simulink model "pid_aw_lazo"  (R2025b)
settings: Solver=FixedStepDiscrete  StartTime=0.0  StopTime=10  FixedStep=Ts  RelTol=1e-3
PreLoadFcn:
  | Ts = 1e-3; tau = 0.01; ad = exp(-Ts/tau); bd = 1 - ad;
undefined symbols (not defined in the file or in its folder): dspblkCoreblockFVToolHelper, gcbh
settings Model: SILPILSystemUnderTest=refmodels  CodeVerificationMode=processor-in-the-loop (pil)  Creator=jnune  LastModifiedBy=jnune
settings OptimizationCC: DefaultParameterBehavior=Inlined  EnhancedBackFolding=on  PassReuseOutputArgsAs=Individual arguments  ZeroExternalMemoryAtStartup=off  ZeroInternalMemoryAtStartup=off  MaxStackSize=64  OptimizeBlockOrder=speed  DifferentSizesBufferReuse=on  OptimizationCustomize=off  EfficientTunableParamExpr=on
settings DebuggingCC: ParameterPrecisionLossMsg=none  ParameterTunabilityLossMsg=error
settings HardwareCC: ProdBitPerPointer=32.0  ProdBitPerSizeT=32.0  ProdBitPerPtrDiffT=32.0  ProdLargestAtomicInteger=Long  ProdLargestAtomicFloat=Double  ProdWordSize=32.0  ProdLongLongMode=on  ProdHWDeviceType=ARM Compatible->ARM Cortex-M
settings SFSimCC: MATLABDynamicMemAlloc=off
settings RTWCC: SystemTargetFile=ert.tlc  HardwareBoard=STM32 Nucleo F767ZI  TemplateMakefile=ert_default_tmf  Toolchain=GNU Tools for ARM Embedded Processors  CodeExecutionProfiling=on  CodeProfilingSaveOptions=AllData  Description=Embedded Coder
settings CodeAppCC: ForceParamTrailComments=on  IgnoreCustomStorageClasses=off  OperatorAnnotations=on  SimulinkDataObjDesc=on  SFDataObjDesc=on  InsertBlockDesc=on
settings ERTTargetCC: ExtModeTransport=3.0  ExtModeStaticAlloc=on  ExtModeStaticAllocSize=2000.0  ExtModeMexFile=ext_xcp  ExtModeIntrfLevel=Level2 - Open  TargetLangStandard=C99 (ISO)

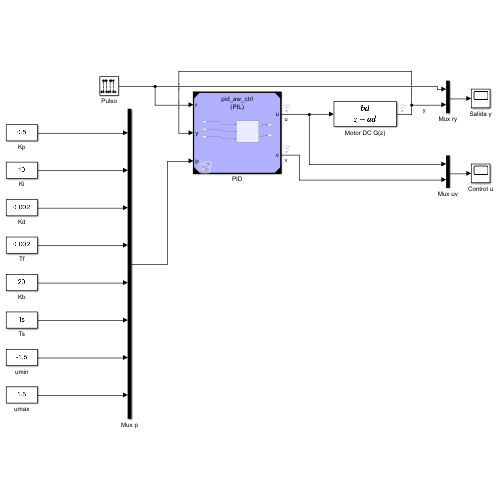
[thumbnail: Simulink's stored preview of the top-level diagram]
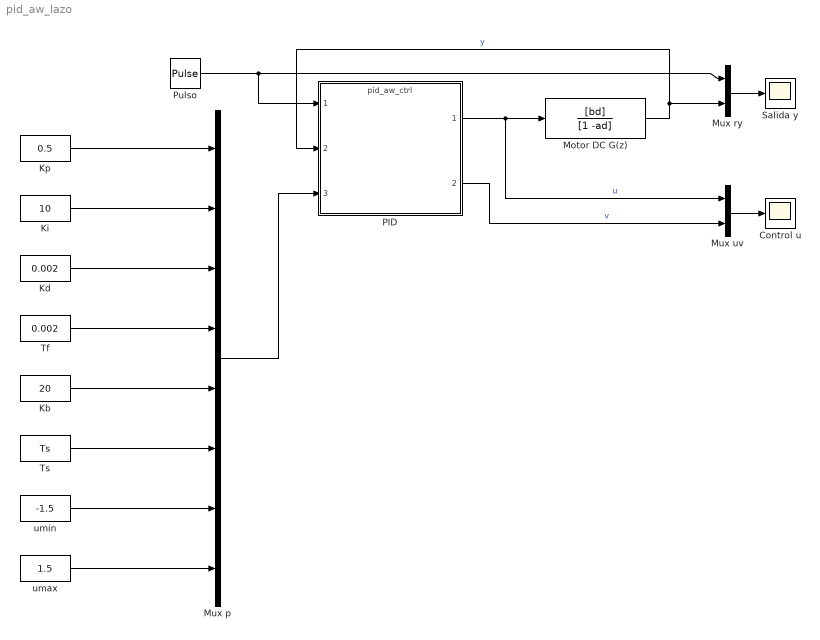
== system pid_aw_lazo ==
  Control u : Scope
      settings: ActiveDisplayYMinimum=-1  ActiveDisplayYMaximum=1
  Kb : Constant  Value=20  SampleTime=Ts
  Kd : Constant  Value=0.002  SampleTime=Ts
  Ki : Constant  Value=10  SampleTime=Ts
  Kp : Constant  Value=0.5  SampleTime=Ts
  Motor DC G(z) : DiscreteTransferFcn  LoadFcn=dspblkCoreblockFVToolHelper(gcbh,'load');  Numerator=[bd]  Denominator=[1 -ad]  SampleTime=Ts
      settings: CopyFcn=dspblkCoreblockFVToolHelper(gcbh,'copy');  DeleteFcn=dspblkCoreblockFVToolHelper(gcbh,'close');  ModelCloseFcn=dspblkCoreblockFVToolHelper(gcbh,'close');  PreSaveFcn=dspblkCoreblockFVToolHelper(gcbh,'presave');  PostSaveFcn=dspblkCoreblockFVToolHelper(gcbh,'postsave');  CloseFcn=dspblkCoreblockFVToolHelper(gcbh,'close');
  Mux p : Mux  Inputs=8
  Mux ry : Mux  Inputs=2
  Mux uv : Mux  Inputs=2
  PID : ModelReference  ModelNameDialog=pid_aw_ctrl  SimulationMode=Processor-in-the-loop (PIL)  ModelReferenceVersion=1.1
  Pulso : DiscretePulseGenerator  Period=2000  PulseWidth=1000  PhaseDelay=100  SampleTime=Ts
  Salida y : Scope
      settings: ActiveDisplayYMinimum=-0.12499999999999997  ActiveDisplayYMaximum=1.125
  Tf : Constant  Value=0.002  SampleTime=Ts
  Ts : Constant  Value=Ts  SampleTime=Ts
  umax : Constant  Value=1.5  SampleTime=Ts
  umin : Constant  Value=-1.5  SampleTime=Ts
  wires:
  Kp/1 -> Mux p/1
  Ki/1 -> Mux p/2
  Kd/1 -> Mux p/3
  Tf/1 -> Mux p/4
  Ts/1 -> Mux p/6
  umin/1 -> Mux p/7
  umax/1 -> Mux p/8
  Kb/1 -> Mux p/5
  Pulso/1 -> PID/1, Mux ry/1
  Mux p/1 -> PID/3
  PID/1 -> Motor DC G(z)/1, Mux uv/1  "u"
  PID/2 -> Mux uv/2  "v"
  Motor DC G(z)/1 -> PID/2, Mux ry/2  "y"
  Mux ry/1 -> Salida y/1
  Mux uv/1 -> Control u/1
